simulink model "openloop_model_LQ_LQE"  (R2026a)
settings: Solver=VariableStepAuto
undefined symbols (not defined in the file): A, B, C, dspblkCoreblockFVToolHelper, gcbh, K, Ke, Kp, MIO, Mk, National_Instruments, Nbar, PCI
libraries: sldrtlib x3
settings Model: Creator=aluno  LastModifiedBy=aluno

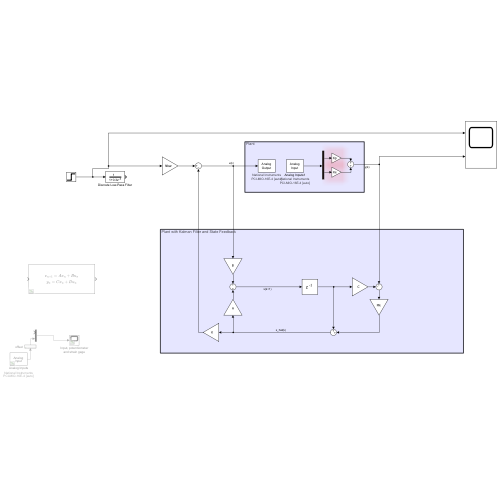
[thumbnail: Simulink's stored preview of the top-level diagram]
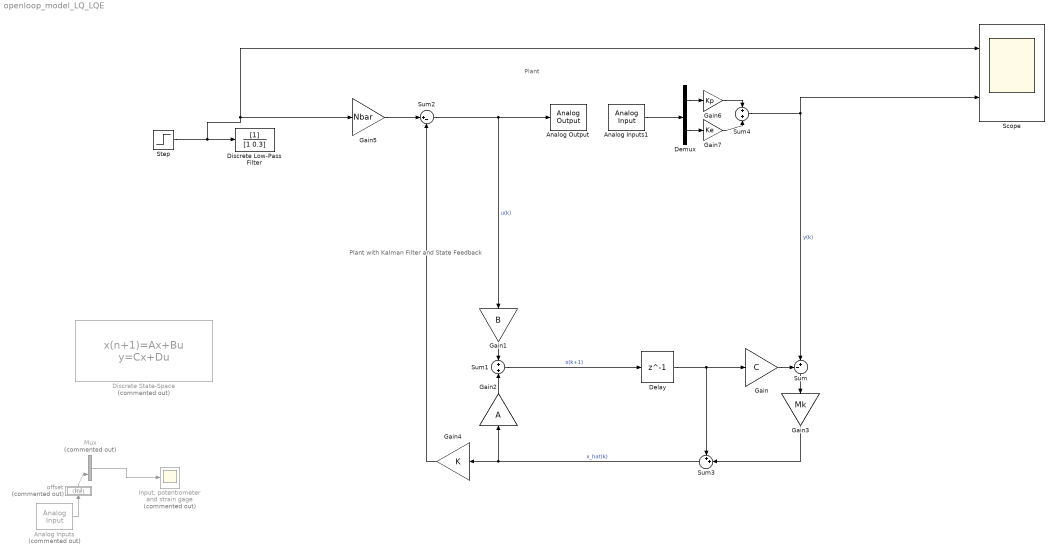
== system openloop_model_LQ_LQE ==
  note: Plant
  note: Plant with Kalman Filter and State Feedback
  Analog Inputs : sldrtlib/Analog Input  Commented=on  SampleTime=0.02  MaxMissedTicks=1000  ShowMissedTicks=off  YieldWhenWaiting=off  DrvName=National_Instruments/PCI-MIO-16E-4  DrvAddress=4294967295  DrvOptions=[0 0 0 0 0 0]  Channels=1:4  RangeMode=1  VoltRange=1  DataType=1
      settings: AttributesFormatString=National Instruments\nPCI-MIO-16E-4 [auto]
  Analog Inputs1 : sldrtlib/Analog Input  SampleTime=0.02  MaxMissedTicks=1000  ShowMissedTicks=off  YieldWhenWaiting=off  DrvName=National_Instruments/PCI-MIO-16E-4  DrvAddress=4294967295  DrvOptions=[0 0 0 0 0 0]  Channels=1:2  RangeMode=1  VoltRange=1  DataType=1
      settings: AttributesFormatString=National Instruments\nPCI-MIO-16E-4 [auto]
  Analog Output : sldrtlib/Analog Output  SampleTime=0.02  MaxMissedTicks=1000  ShowMissedTicks=off  YieldWhenWaiting=off  DrvName=National_Instruments/PCI-MIO-16E-4  DrvAddress=4294967295  DrvOptions=[0 0 0 0 0 0]  Channels=1  RangeMode=1  VoltRange=1  InitialValue=0  FinalValue=0
      settings: AttributesFormatString=National Instruments\nPCI-MIO-16E-4 [auto]
  Delay : Delay  DelayLength=1  InputProcessing=Columns as channels (frame based)
  Demux : Demux  Outputs=2
  Discrete Low-Pass Filter : DiscreteFilter  LoadFcn=dspblkCoreblockFVToolHelper(gcbh,'load');  Denominator=[1 0.3]
      settings: CopyFcn=dspblkCoreblockFVToolHelper(gcbh,'copy');  DeleteFcn=dspblkCoreblockFVToolHelper(gcbh,'close');  ModelCloseFcn=dspblkCoreblockFVToolHelper(gcbh,'close');  PreSaveFcn=dspblkCoreblockFVToolHelper(gcbh,'presave');  PostSaveFcn=dspblkCoreblockFVToolHelper(gcbh,'postsave');  CloseFcn=dspblkCoreblockFVToolHelper(gcbh,'close');
  Discrete State-Space : DiscreteStateSpace  Commented=on  A=A  B=B  C=C  D=0  SampleTime=-1
  Gain : Gain  Gain=C
  Gain1 : Gain  Gain=B
  Gain2 : Gain  Gain=A
  Gain3 : Gain  Gain=Mk
  Gain4 : Gain  Gain=K
  Gain5 : Gain  Gain=Nbar
  Gain6 : Gain  Gain=Kp
  Gain7 : Gain  Gain=Ke
  "Input, potentiometer and strain gage" : Scope  Commented=on
      settings: DataLoggingSaveFormat=Array
  Mux : Mux  Commented=on  Inputs=2
  Scope : Scope  NumInputPorts=2
  Step : Step  SampleTime=0
  Sum : Sum  Inputs=-+|
  Sum1 : Sum  Inputs=+|+
  Sum2 : Sum  Inputs=|+-
  Sum3 : Sum  Inputs=++|
  Sum4 : Sum  Inputs=+|+
  offset : Subsystem  Commented=on
  wires:
  Gain/1 -> Sum/1
  Delay/1 -> Sum3/1, Gain/1
  Sum1/1 -> Delay/1  "x(k+1)"
  Gain1/1 -> Sum1/1
  Gain2/1 -> Sum1/2
  Sum2/1 -> Analog Output/1, Gain1/1  "u(k)"
  Sum/1 -> Gain3/1
  Gain3/1 -> Sum3/2
  Sum3/1 -> Gain2/1, Gain4/1  "x_hat(k)"
  Gain4/1 -> Sum2/2
  Gain5/1 -> Sum2/1
  offset/1(Out1) -> Mux/2
  Analog Inputs/1 -> offset/1(In1)
  Step/1 -> Gain5/1, Scope/1, Discrete Low-Pass Filter/1
  Mux/1 -> "Input, potentiometer and strain gage"/1
  Analog Inputs1/1 -> Demux/1
  Demux/1 -> Gain6/1
  Demux/2 -> Gain7/1
  Sum4/1 -> Sum/2, Scope/2  "y(k)"
  Gain6/1 -> Sum4/1
  Gain7/1 -> Sum4/2

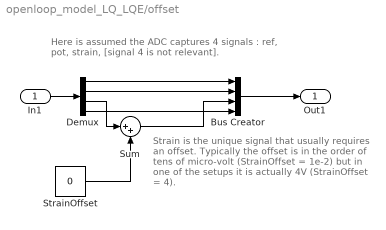
== system openloop_model_LQ_LQE/offset ==
  note: Strain is the unique signal that usually requires an offset. Typically the offset is in the order of tens of micro-volt (StrainOffset = 1e-2) but in one of the setups it is actually 4V (StrainOffset = 4).
  note: Here is assumed the ADC captures 4 signals :
      | ref, pot, strain, [signal 4 is not relevant].
  In1 : Inport
  Bus Creator : BusCreator  Inputs=4
  Demux : Demux
  StrainOffset : Constant  Value=0
  Sum : Sum  Inputs=|++
  Out1 : Outport
  wires:
  In1/1 -> Demux/1
  Bus Creator/1 -> Out1/1
  Demux/1 -> Bus Creator/1
  Demux/2 -> Bus Creator/2
  Demux/4 -> Bus Creator/4
  Demux/3 -> Sum/1
  Sum/1 -> Bus Creator/3
  StrainOffset/1 -> Sum/2
